simulink model "signal_generator_comparison"  (R2025a)
settings: Solver=VariableStepAuto  StartTime=0.0  StopTime=200  RelTol=1e-3
libraries: simulink x1
settings Model: Creator=e82540u  LastModifiedBy=e82540u

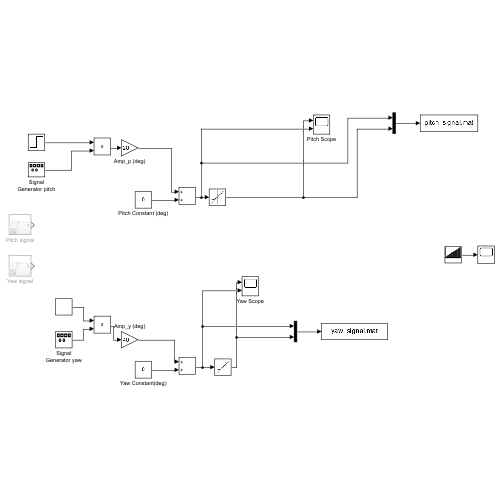
[thumbnail: Simulink's stored preview of the top-level diagram]
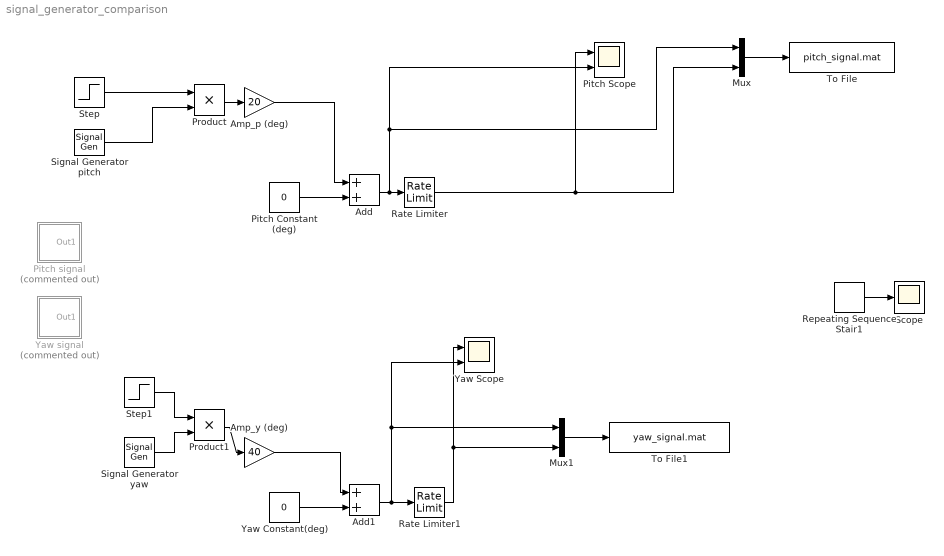
== system signal_generator_comparison ==
  Add : Sum
  Add1 : Sum
  Amp_p (deg) : Gain  Gain=20
  Amp_y (deg) : Gain  Gain=40
  Mux : Mux  Inputs=2
  Mux1 : Mux  Inputs=2
  Pitch Constant (deg) : Constant  Value=0
  Pitch Scope : Scope  NumInputPorts=2
      settings: ActiveDisplayYMinimum=-60.25223030602023  ActiveDisplayYMaximum=48.891499113076627
  Pitch signal : Subsystem  Commented=on
  Product : Product
  Product1 : Product
  Rate Limiter : RateLimiter  RisingSlewLimit=20  FallingSlewLimit=-20  SampleTimeMode=inherited
  Rate Limiter1 : RateLimiter  RisingSlewLimit=20  FallingSlewLimit=-20  SampleTimeMode=inherited
  Repeating Sequence Stair1 : simulink/Sources/Repeating Sequence Stair  OutValues=reshape([zeros(1,20); 1:20], 1, [])  tsamp=5  OutMin=[]  OutMax=[]  OutDataTypeStr=double  OutputDataTypeScalingMode=double  OutDataType=fixdt(0,8)  ConRadixGroup=Best Precision: Vector-wise  OutScaling=2^-12
  Scope : Scope
      settings: ActiveDisplayYMinimum=-2.4999999999999996  ActiveDisplayYMaximum=22.5  DataLoggingVariableName=ScopeData2
  Signal Generator pitch : SignalGenerator  WaveForm=square  Frequency=0.1
  Signal Generator yaw : SignalGenerator  WaveForm=square  Frequency=0.04
  Step : Step  SampleTime=0
  Step1 : Step  SampleTime=0
  To File : ToFile  Filename=pitch_signal.mat  MatrixName=pitch
  To File1 : ToFile  Filename=yaw_signal.mat  MatrixName=yaw
  Yaw Constant(deg) : Constant  Value=0
  Yaw Scope : Scope  NumInputPorts=2
      settings: ActiveDisplayYMinimum=-21.41521791771828  ActiveDisplayYMaximum=93.185697972333443
  Yaw signal : Subsystem  Commented=on
  wires:
  Pitch Constant (deg)/1 -> Add/2
  Yaw Constant(deg)/1 -> Add1/2
  Signal Generator pitch/1 -> Product/2
  Signal Generator yaw/1 -> Product1/2
  Add/1 -> Mux/1, Pitch Scope/2, Rate Limiter/1
  Mux/1 -> To File/1
  Mux1/1 -> To File1/1
  Add1/1 -> Mux1/1, Yaw Scope/2, Rate Limiter1/1
  Rate Limiter/1 -> Mux/2, Pitch Scope/1
  Rate Limiter1/1 -> Mux1/2, Yaw Scope/1
  Step/1 -> Product/1
  Product/1 -> Amp_p (deg)/1
  Step1/1 -> Product1/1
  Product1/1 -> Amp_y (deg)/1
  Amp_p (deg)/1 -> Add/1
  Amp_y (deg)/1 -> Add1/1
  Repeating Sequence Stair1/1 -> Scope/1

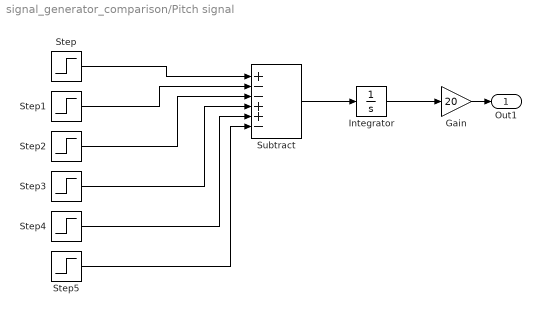
== system signal_generator_comparison/Pitch signal ==
  Gain : Gain  Gain=20
  Integrator : Integrator
  Step : Step  SampleTime=5
  Step1 : Step  SampleTime=6
  Step2 : Step  SampleTime=10
  Step3 : Step  SampleTime=12
  Step4 : Step  SampleTime=15
  Step5 : Step  SampleTime=17
  Subtract : Sum  Inputs=+--++-
  Out1 : Outport
  wires:
  Gain/1 -> Out1/1
  Step3/1 -> Subtract/4
  Step/1 -> Subtract/1
  Subtract/1 -> Integrator/1
  Step4/1 -> Subtract/5
  Step5/1 -> Subtract/6
  Integrator/1 -> Gain/1
  Step1/1 -> Subtract/2
  Step2/1 -> Subtract/3

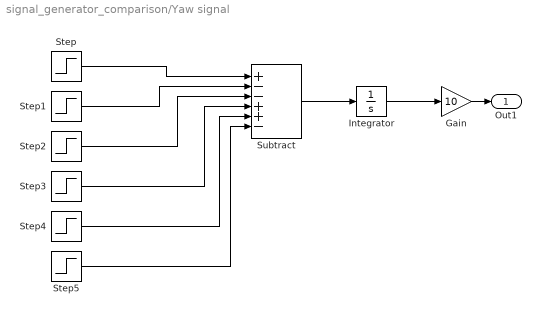
== system signal_generator_comparison/Yaw signal ==
  Gain : Gain  Gain=10
  Integrator : Integrator
  Step : Step  After=2  SampleTime=12.5
  Step1 : Step  After=2  SampleTime=13.5
  Step2 : Step  After=2  SampleTime=25
  Step3 : Step  After=2  SampleTime=27
  Step4 : Step  After=2  SampleTime=47.5
  Step5 : Step  After=2  SampleTime=49.5
  Subtract : Sum  Inputs=+--++-
  Out1 : Outport
  wires:
  Gain/1 -> Out1/1
  Step3/1 -> Subtract/4
  Step/1 -> Subtract/1
  Subtract/1 -> Integrator/1
  Step4/1 -> Subtract/5
  Step5/1 -> Subtract/6
  Integrator/1 -> Gain/1
  Step1/1 -> Subtract/2
  Step2/1 -> Subtract/3
